simulink model "DABThermalAnalysisWithCustomMOSFET"  (R2026a)
settings: Solver=ode23t  StopTime=0.06  MaxStep=1e-5  AbsTol=1e-3
PreLoadFcn:
  | DABThermalAnalysisWithCustomMOSFETInputParameters;
model workspace (MAT data in the model file):
  ConverterKey = "DAB"
undefined symbols (not defined in the file): DAB, DABController, DABDesign, DiscIntNeverNeededParam, M1p, M1s, M2p, M2s, M3p, M3s, M4p, M4s
libraries: ee_lib x21, nesl_utility x16, fl_lib x11, slpidlib x4, simulink_extras x1
(part 1 of 2)
settings Model: SimulationMode=accelerator  Creator=vsolaise  LastModifiedBy=vsolaise
settings SimscapeCC: SimscapeNominalValues="[{\"value\":\"1\",\"unit\":\"A\"},{\"value\":\"1\",\"unit\":\"bar\"},{\"value\":\"1\",\"unit\":\"cm^2\"},{\"value\":\"1\",\"unit\":\"cm^3/s\"},{\"value\":\"1\",\"unit\":\"kJ/kg\"},{\"value\":\"1\",\"unit\":\"kW\"},{\"value\":\"1\",\"unit\":\"l\"},{\"value\":\"1\",\"unit\":\"N\"},{\"value\":\"1\",\"unit\":\"N*m\"},{\"value\":\"1\",\"unit\":\"V\"}]"  SimscapeLogName=simlogDABThermal  SimscapeLogDataHistory=5000.0

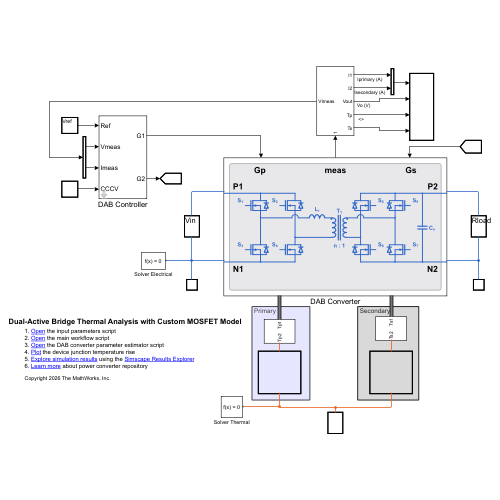
[thumbnail: Simulink's stored preview of the top-level diagram]
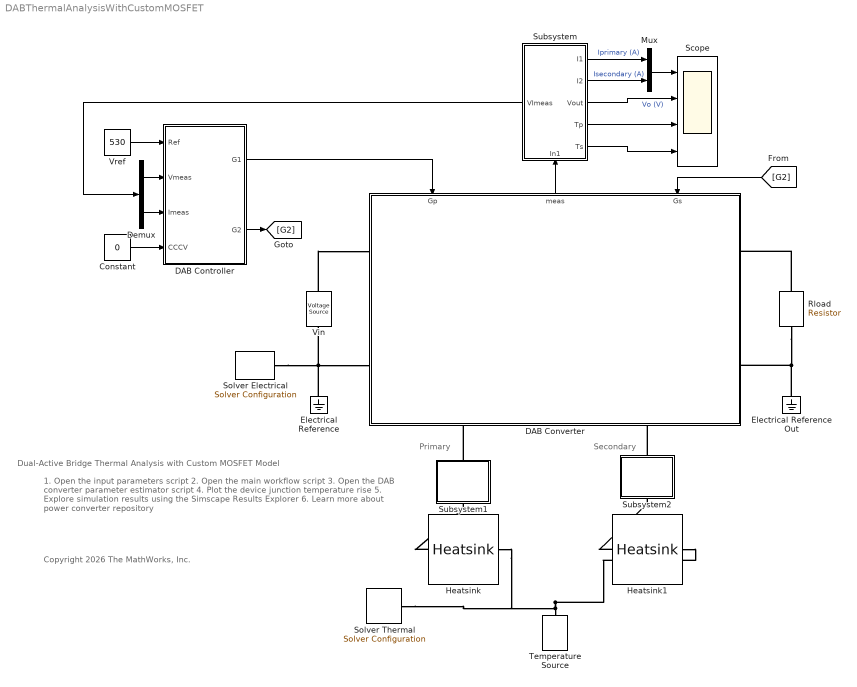
== system DABThermalAnalysisWithCustomMOSFET ==
  note: Secondary
  note: Primary
  note: Copyright 2026 The MathWorks, Inc.
  note: Dual-Active Bridge Thermal Analysis with Custom MOSFET Model
  note: 1. Open the input parameters script
      | 2. Open the main workflow script
      | 3. Open the DAB converter parameter estimator script
      | 4. Plot the device junction temperature rise
      | 5. Explore simulation results using the Simscape Results Explorer
      | 6. Learn more about power converter repository
  Constant : Constant  Value=0
  DAB Controller : Subsystem  mask(Dual Active Bridge Phase-Shift Controller){outputSelect=Gate Signals, cntrlSelect=PI controller (Continuous), Vbase=DABDesign.V2nom.value, Pbase=DABDesign.ratedPower.value, Fsw=DABDesign.switchingFrequency.value, Tdead=DABDesign.deadTime.value, primaryGateVoltage=DABController.gateVoltage, secondaryGateVoltage=DABController.gateVoltage, Ts=DABController.sampleTime, phaseShiftMax=DABController.phaseShiftMax, phaseShiftMin=DABController.phaseShiftMin, Kp=DABController.currentLoopProportionalGain, Ki=DABController.currentLoopIntegralGain, Kpv=DABController.voltageLoopProportionalGain, Kiv=DABController.voltageLoopIntegralGain}
      mask prompts: outputSelect "Output mode"; cntrlSelect "Controller type"; Vbase "Nominal output voltage (V)"; Pbase "Nominal power (W)"; Fsw "Switching frequency (Hz)"; Tdead "Dead time (s)"; primaryGateVoltage "Primary gate voltage (V)"; secondaryGateVoltage "Secondary gate voltage (V)"; Ts "Sample time (s)"; phaseShiftMax "Max phase shift (rad)"; phaseShiftMin "Min phase shift (rad)"; Kp "Proportional gain (current loop)"; Ki "Integral gain (current loop)"; Kpv "Proportional gain (voltage loop)"; Kiv "Integral gain (voltage loop)"
      mask help:
      | Phase-shift controller for the dual-active-bridge converter, in constant-current or constant-voltage mode. The CCCV input selects which loop runs: CC regulates Imeas against a current reference on Ref, normalized on the base current Pbase/Vbase; CV regulates Vmeas against a voltage reference on Ref, normalized on Vbase. Either PI drives the bridge-to-bridge phase shift, limited by phaseShiftMin and phaseShiftMax. Offers PI controllers in continuous or discrete form, with selectable phase shift or gate signal output.
      |
      | Outputs G1 and G2 are the primary and secondary bridge gate vectors, at the levels set by primaryGateVoltage and secondaryGateVoltage. In Phase Shift (rad) mode both outputs instead carry the phase shift itself, for use with an averaged plant.
      mask init:
      | dabControllerMaskInit(gcb);
      mask TypeOptions outputSelect: Gate Signals | Phase Shift (rad)
      mask Callback outputSelect: selectDABControllerOutputMode(gcb);
      mask TypeOptions cntrlSelect: PI controller (Continuous) | PI controller (Discrete)
      mask Callback cntrlSelect: selectDABControllerType(gcb);
      mask DialogControl Container5 Prompt: DAB Converter Parameter
      mask DialogControl ControllerPanel Prompt: Current Controller
      mask DialogControl VoltageLoopPanel Prompt: Voltage Controller
  DAB Converter : Subsystem
      settings: CopyFcn="set_param(gcbh,\"LinkStatus\",\"none\");"  PortSchema="{\"entries\":[{\"content\":{\"sides\":[{\"content\":{\"connectorIds\":[\"LConn1\",\"LConn2\"]},\"type\":\"ConnectorPlacement.EquallySpacedRectSide\",\"uuid\":\"033d868c-c914-47ac-88c6-7cc8bbca37ec\"},{\"content\":{\"connectorIds\":[\"RConn1\",\"RConn2\"],\"side\":\"RIGHT\"},\"type\":\"ConnectorPlacement.EquallySpacedRectSide\",\"uuid\":\"51ef52ad-95d3-4257-8134-5dc220f84f04\"},{\"content\":{\"connectorIds\":[\"In1\",\"Out1\",\"In2\"],\"side\":\"TOP\"},\"type\":\"ConnectorPlacement.EquallySpacedRectSide\",\"uuid\":\"aa7ed817-9ae7-4471-a537-30f60ddc8f94\"},{\"content\":{\"connectorIds\":[\"RConn3\",\"RConn4\"],\"side\":\"BOTTOM\"},\"type\":\"ConnectorPlacement.EquallySpacedRectSide\",\"uuid\":\"1eb7cc02-5c97-4e68-b623-57bf124e9704\"}]},\"type\":\"ConnectorPlacement.EquallySpacedConnector\",\"uuid\":\"613f6d24-3cc9-4a3f-99a5-466a272a8233\"}],\"packageUris\":[\"http://schema.mathworks.com/mf0/Connector/R2020b\"],\"version\":\"1.0\"}"
      mask Display: image('DABConverterIcon.svg');
  Demux : Demux  Outputs=2
  Electrical Reference : fl_lib/Electrical/Electrical Elements/Electrical Reference
  Electrical Reference Out : fl_lib/Electrical/Electrical Elements/Electrical Reference
  Heatsink : ee_lib/Passive/Thermal/Heatsink  parameterization=ee.enum.passive.thermal.heatsinkParam.datasheet  convection=ee.enum.passive.thermal.heatsinkConvection.natural  T_vec_Q=[10, 30, 50, 70, 90] K  v_vec_Q=[0, 1, 2, 3] m/s  Q_TLU1=[10, 30, 50, 70, 90]/DAB.HeatsinkPri.sinkToAmbientResistance W  Q_TLU2=[6.1, 18.8, 22.8, 25.7; 23.6, 61.1, 73, 81.5; 44.5, 106.4, 125.9, 140.1; 67.5, 153.5, 180.7, 200.3; 92.3, 202.1, 236.9, 262] W  T_vec_h=[10, 30, 50, 70, 90] K  v_vec_h=[0, 1, 2, 3] m/s  h_TLU1=[5.4, 7.02, 7.98, 8.68, 9.26] W/(K*m^2)  h_TLU2=[5.4, 17.86, 22.17, 25.41; 7.02, 19.49, 23.8, 27.03; 7.97, 20.44, 24.75, 27.99; 8.68, 21.15, 25.46, 28.69; 9.26, 21.73, 26.04, 29.27] W/(K*m^2)  h_vec=[5, 10, 15, 20, 25, 30] W/(K*m^2)  eff_TLU=[96.97, 94.16, 91.53, 89.08, 86.78, 84.62]  height=38.1e-3 m  thick=6.5e-4 m  depth=139.7e-3 m  gap=9.4e-3 m  num_fins=11  k_fin=237 W/(K*m)  A_total=0.1171 m^2  nu=1.51e-5 m^2/s  alpha=2.07e-5 m^2/s  k_fluid=25e-3 W/(K*m)  beta=3.3e-3 1/K  mass=DAB.HeatsinkPri.mass kg  sp_heat=DAB.HeatsinkPri.specificHeat J/(K*kg)  T_hs_specify=on  T_hs_priority=High  T_hs=DAB.HeatsinkPri.initialTemperature degC  T_hs_nominal_specify=off  T_hs_nominal_value=1  T_hs_nominal_unit=K  Q_A_specify=off  Q_A_priority=None  Q_A=0 W  Q_A_nominal_specify=off  Q_A_nominal_value=1  Q_A_nominal_unit=W  Q_C_specify=off  Q_C_priority=None  Q_C=0 W  Q_C_nominal_specify=off  Q_C_nominal_value=1  Q_C_nominal_unit=W
  Heatsink1 : ee_lib/Passive/Thermal/Heatsink  parameterization=ee.enum.passive.thermal.heatsinkParam.datasheet  convection=ee.enum.passive.thermal.heatsinkConvection.natural  T_vec_Q=[10, 30, 50, 70, 90] K  v_vec_Q=[0, 1, 2, 3] m/s  Q_TLU1=[10, 30, 50, 70, 90]/DAB.HeatsinkSec.sinkToAmbientResistance W  Q_TLU2=[6.1, 18.8, 22.8, 25.7; 23.6, 61.1, 73, 81.5; 44.5, 106.4, 125.9, 140.1; 67.5, 153.5, 180.7, 200.3; 92.3, 202.1, 236.9, 262] W  T_vec_h=[10, 30, 50, 70, 90] K  v_vec_h=[0, 1, 2, 3] m/s  h_TLU1=[5.4, 7.02, 7.98, 8.68, 9.26] W/(K*m^2)  h_TLU2=[5.4, 17.86, 22.17, 25.41; 7.02, 19.49, 23.8, 27.03; 7.97, 20.44, 24.75, 27.99; 8.68, 21.15, 25.46, 28.69; 9.26, 21.73, 26.04, 29.27] W/(K*m^2)  h_vec=[5, 10, 15, 20, 25, 30] W/(K*m^2)  eff_TLU=[96.97, 94.16, 91.53, 89.08, 86.78, 84.62]  height=38.1e-3 m  thick=6.5e-4 m  depth=139.7e-3 m  gap=9.4e-3 m  num_fins=11  k_fin=237 W/(K*m)  A_total=0.1171 m^2  nu=1.51e-5 m^2/s  alpha=2.07e-5 m^2/s  k_fluid=25e-3 W/(K*m)  beta=3.3e-3 1/K  mass=DAB.HeatsinkSec.mass kg  sp_heat=DAB.HeatsinkSec.specificHeat J/(K*kg)  T_hs_specify=on  T_hs_priority=High  T_hs=DAB.HeatsinkSec.initialTemperature degC  T_hs_nominal_specify=off  T_hs_nominal_value=1  T_hs_nominal_unit=K  Q_A_specify=off  Q_A_priority=None  Q_A=0 W  Q_A_nominal_specify=off  Q_A_nominal_value=1  Q_A_nominal_unit=W  Q_C_specify=off  Q_C_priority=None  Q_C=0 W  Q_C_nominal_specify=off  Q_C_nominal_value=1  Q_C_nominal_unit=W
  Mux : Mux  Inputs=2
  Rload : fl_lib/Electrical/Electrical Elements/Resistor  R=40 Ohm  i_specify=off  i_priority=None  i=0 A  i_nominal_specify=off  i_nominal_value=1  i_nominal_unit=A  v_specify=off  v_priority=None  v=0 V  v_nominal_specify=off  v_nominal_value=1  v_nominal_unit=V
  Scope : Scope  NumInputPorts=4
      settings: Title=Transformer current  ActiveDisplayYMinimum=-32.189332854725691  ActiveDisplayYMaximum=31.187175123208139  YLabel=Current (A)
  Solver Electrical : nesl_utility/Solver Configuration  PhysicalDomain=network_engine_domain  SubClassName=solver  LeftPortType=input  RightPortType=generic  Tones=[]  Harmonics=[]  SimulateNoise=off  Profile=off  UseLocalSampling=off  EnableSwitchedLinearOptims=on  FrequencyDomain=off  UseCCode=off  RelTol=0.001  AbsTol=0.001  MinStep=1e-09  ToWorkspace=off  RevertToSquareIcSolve=off  NumHomotopyIterations=100  PhasorMode=off  PhasorModeNumHarmonics=1  ConsistencySolver=NEWTON_XTOL_AFTER_FTOL  CanonicalOrdering=UNORDERED  OptimizeIntermediates=UNOPTIMIZED  IndexReductionMethod=DerivativeReplacement  DoDC=off  ResidualTolerance=1e-09  ConsistencyTolSource=GLOBAL  ConsistencyAbsTol=0.001  ConsistencyRelTol=0.001  ConsistencyTolFactor=0.001  UseLocalSolver=on  LocalSolverChoice=NE_PARTITIONING_ADVANCER  ResolveIndetEquations=on  FunctionEvalNumThread=1  LocalSolverSampleTime=1.5e-7  DoFixedCost=off  MaxNonlinIter=20  MaxModeIter=2  ComputeImpulses=off  ImpulseIterations=2  LinearAlgebra=auto  LinearAlgebraNumThread=0  EquationFormulation=NE_TIME_EF  DelaysMemoryBudget=1024  AutomaticFiltering=on  FilteringTimeConstant=0.001  PartitionStorageMethod=AS_NEEDED  PartitionMemoryBudget=1024  PartitionMethod=ROBUST  MultibodyUseLocalSolver=off  MultibodyLocalSolverChoice=ODE1  MultibodyLocalSolverSampleTime=0.001
  Solver Thermal : nesl_utility/Solver Configuration  PhysicalDomain=network_engine_domain  SubClassName=solver  LeftPortType=input  RightPortType=generic  Tones=[]  Harmonics=[]  SimulateNoise=off  Profile=off  UseLocalSampling=off  EnableSwitchedLinearOptims=on  FrequencyDomain=off  UseCCode=off  RelTol=0.001  AbsTol=0.001  MinStep=1e-09  ToWorkspace=off  RevertToSquareIcSolve=off  NumHomotopyIterations=100  PhasorMode=off  PhasorModeNumHarmonics=1  ConsistencySolver=NEWTON_XTOL_AFTER_FTOL  CanonicalOrdering=CANONICAL  OptimizeIntermediates=OPTIMIZED  IndexReductionMethod=DerivativeReplacement  DoDC=off  ResidualTolerance=1e-09  ConsistencyTolSource=GLOBAL  ConsistencyAbsTol=0.001  ConsistencyRelTol=0.001  ConsistencyTolFactor=0.001  UseLocalSolver=on  LocalSolverChoice=NE_BACKWARD_EULER_ADVANCER  ResolveIndetEquations=on  FunctionEvalNumThread=1  LocalSolverSampleTime=0.00001  DoFixedCost=off  MaxNonlinIter=3  MaxModeIter=2  ComputeImpulses=off  ImpulseIterations=2  LinearAlgebra=auto  LinearAlgebraNumThread=0  EquationFormulation=NE_TIME_EF  DelaysMemoryBudget=1024  AutomaticFiltering=on  FilteringTimeConstant=0.001  PartitionStorageMethod=AS_NEEDED  PartitionMemoryBudget=1024  PartitionMethod=ROBUST  MultibodyUseLocalSolver=off  MultibodyLocalSolverChoice=ODE1  MultibodyLocalSolverSampleTime=0.001
  Subsystem : Subsystem
      settings: PortSchema="{\"entries\":[{\"content\":{\"sides\":[{\"content\":{\"connectorIds\":[\"Out6\"]},\"type\":\"ConnectorPlacement.EquallySpacedRectSide\",\"uuid\":\"f2b899f7-a6f0-4063-b280-75fc43e532d5\"},{\"content\":{\"connectorIds\":[\"Out1\",\"Out2\",\"Out3\",\"Out4\",\"Out5\"],\"side\":\"RIGHT\"},\"type\":\"ConnectorPlacement.EquallySpacedRectSide\",\"uuid\":\"5de70531-a79e-4c62-9cd6-16ab34a78e6e\"},{\"content\":{\"side\":\"TOP\"},\"type\":\"ConnectorPlacement.EquallySpacedRectSide\",\"uuid\":\"e5bc4a57-59c4-404a-a3d7-aeb4f7590bd8\"},{\"content\":{\"connectorIds\":[\"In1\"],\"side\":\"BOTTOM\"},\"type\":\"ConnectorPlacement.EquallySpacedRectSide\",\"uuid\":\"d1dcebc2-7af2-4d54-9158-2e062e509fbc\"}]},\"type\":\"ConnectorPlacement.EquallySpacedConnector\",\"uuid\":\"ad567749-1bde-47d1-aaf1-1f8d8a2cad80\"}],\"packageUris\":[\"http://schema.mathworks.com/mf0/Connector/R2020b\"],\"version\":\"1.0\"}"
  Subsystem1 : Subsystem
  Subsystem2 : Subsystem
  Temperature Source : fl_lib/Thermal/Thermal Sources/Temperature Source  temperature=298.15 K
  Vin : ee_lib/Sources/Voltage Source  dc_voltage=770 V  ac_voltage=0 V  ac_shift=0 rad  ac_frequency=60 Hz  noise_mode=ee.enum.sources.noise.Disabled  PSD=0 V^2/Hz  sample_time=1e-3 s  repeatability=ee.enum.sources.repeatability.NotRepeatable  user_seed=0  auto_seed=1556750757  i_specify=off  i_priority=None  i=0 A  i_nominal_specify=off  i_nominal_value=1  i_nominal_unit=A  v_specify=off  v_priority=None  v=0 V  v_nominal_specify=off  v_nominal_value=1  v_nominal_unit=V
  Vref : Constant  Value=530
  wires:
  DAB Controller/2(G2) -> [G2]
  Constant/1 -> DAB Controller/4(CCCV)
  Subsystem/1(I1) -> Mux/1  "Iprimary (A)"
  Subsystem/2(I2) -> Mux/2  "Isecondary (A)"
  DAB Converter/1(meas) -> Subsystem/1(In1)
  Vref/1 -> DAB Controller/1(Ref)
  Demux/2 -> DAB Controller/3(Imeas)
  Demux/1 -> DAB Controller/2(Vmeas)
  Subsystem/6(VImeas) -> Demux/1
  DAB Controller/1(G1) -> DAB Converter/1(Gp)
  [G2] -> DAB Converter/2(Gs)
  Mux/1 -> Scope/1
  Subsystem/3(Vout) -> Scope/2  "Vo (V)"
  Subsystem/4(Tp) -> Scope/3
  Subsystem/5(Ts) -> Scope/4
  connections:
  Vin/LConn1 -- DAB Converter/LConn1
  Rload/LConn1 -- DAB Converter/RConn1
  Solver Electrical/RConn1 -- Electrical Reference/LConn1 -- Vin/RConn1 -- DAB Converter/LConn2
  Rload/RConn1 -- Electrical Reference Out/LConn1 -- DAB Converter/RConn2
  Temperature Source/LConn1 -- Heatsink1/LConn1 -- Heatsink/LConn1 -- Solver Thermal/RConn1
  Subsystem2/RConn1 -- DAB Converter/RConn4
  Subsystem1/RConn1 -- DAB Converter/RConn3
  Heatsink1/RConn1 -- Subsystem2/LConn1
  Heatsink/RConn1 -- Subsystem1/LConn1

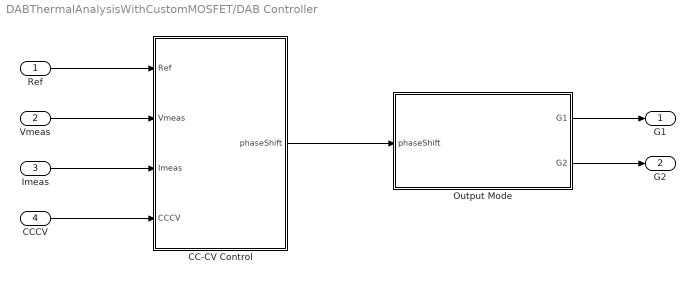
== system DABThermalAnalysisWithCustomMOSFET/DAB Controller ==
  Ref : Inport
  Vmeas : Inport  Port=2
  Imeas : Inport  Port=3
  CCCV : Inport  Port=4
  CC-CV Control : Subsystem
  Output Mode : Subsystem  Variant=on  VariantControlMode=label  LabelModeActiveChoice=PWMSignal
  G1 : Outport
  G2 : Outport  Port=2
  wires:
  CCCV/1 -> CC-CV Control/4(CCCV)
  Imeas/1 -> CC-CV Control/3(Imeas)
  Vmeas/1 -> CC-CV Control/2(Vmeas)
  Ref/1 -> CC-CV Control/1(Ref)
  Output Mode/2(G2) -> G2/1
  Output Mode/1(G1) -> G1/1
  CC-CV Control/1(phaseShift) -> Output Mode/1(phaseShift)

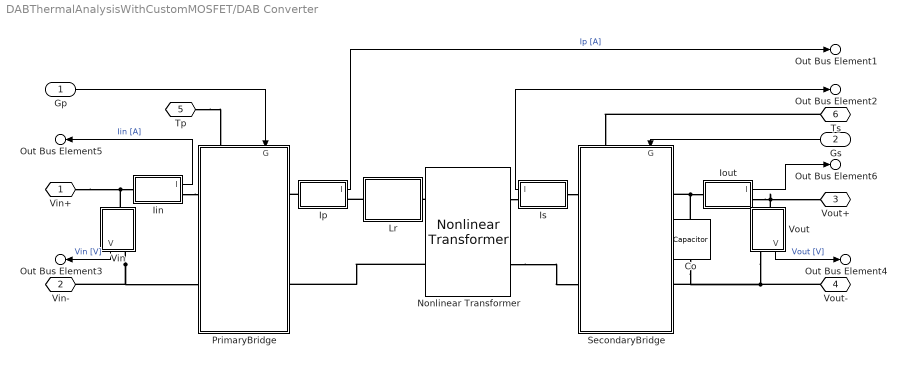
== system DABThermalAnalysisWithCustomMOSFET/DAB Converter ==
  Gp : Inport
  Gs : Inport  Port=2
  Co : ee_lib/Passive/Capacitor  cap_option=ee.enum.passive.capacitor.capOption.const  c=DAB.Co F  Cvec=[1e-05, 1e-06] F  Vvec=[0, 10] V  CV_table_symmetry=ee.enum.passive.capacitor.tableSymmetry.yes  f_vec=[1, 10] kHz  DFext_vec=[.8, 1.2]  enable_C_tol=ee.enum.toleranceApplication.none  averaging_period=0 s  C_tol=5  tol_distribution=ee.enum.toleranceDistribution.uniform  nSigma=4  r=DAB.Rco Ohm  g=0 1/Ohm  enable_operating_limits=ee.enum.enable.no  operating_limit_action=ee.enum.passive.reportOpLim.warn  max_working_voltage_range=[-25, 25] V  power_rating=1 W  maxTemperature=85 degC  thermalEnable=false  thermalMass=1 J/K  i_specify=off  i_priority=None  i=0 A  i_nominal_specify=off  i_nominal_value=1  i_nominal_unit=A  v_specify=off  v_priority=None  v=0 V  v_nominal_specify=off  v_nominal_value=1  v_nominal_unit=V  vc_specify=on  vc_priority=High  vc=DAB.Vco V  vc_nominal_specify=off  vc_nominal_value=1  vc_nominal_unit=V  T_specify=off  T_priority=None  T=298.15 K  T_nominal_specify=off  T_nominal_value=1  T_nominal_unit=K
  Iin : Subsystem
      mask Display: disp('I')
  Iout : Subsystem
      mask Display: disp('I')
  Ip : Subsystem
      mask Display: disp('I')
  Is : Subsystem
      settings: PortSchema="{\"entries\":[{\"content\":{\"sides\":[{\"content\":{\"connectorIds\":[\"Out1\",\"LConn1\"]},\"type\":\"ConnectorPlacement.EquallySpacedRectSide\",\"uuid\":\"da66b42d-39ba-4e5d-9b19-dc680792542d\"},{\"content\":{\"connectorIds\":[\"RConn1\"],\"side\":\"RIGHT\"},\"type\":\"ConnectorPlacement.EquallySpacedRectSide\",\"uuid\":\"9a34d54a-b1f0-405a-82c9-4333c7864e33\"},{\"content\":{\"side\":\"TOP\"},\"type\":\"ConnectorPlacement.EquallySpacedRectSide\",\"uuid\":\"3d98f795-d173-4072-aa84-47617691d0d7\"}]},\"type\":\"ConnectorPlacement.EquallySpacedConnector\",\"uuid\":\"cc1a3107-18f6-4c4b-a82f-56637250e4a4\"}],\"packageUris\":[\"http://schema.mathworks.com/mf0/Connector/R2020b\"],\"version\":\"1.0\"}"
      mask Display: disp('I')
  Lr : Subsystem
  Nonlinear Transformer : ee_lib/Passive/Transformers/Nonlinear Transformer  Nw=DAB.turnsRatio  Nw2=1  winding_param_option=2  Req=0 Ohm  Leq=0 H  R_1=DAB.RLlk1 Ohm  L_1=DAB.Llk1 H  R_2=DAB.RLlk2 Ohm  L_2=DAB.Llk2 H  averaging_period=0 s  R_m=15000 Ohm  parameterization_option=1  H_data=[0, 200, 400, 600, 800, 1000] A/m  B_data=[0, .81, 1.25, 1.42, 1.48, 1.49] T  length_effective=0.2 m  area_effective=2e-4 m^2  L=DAB.Lm H  L_sat=1e-2 H  current_data=[0, .4, .8, 1.2, 1.6, 2] A  magnetic_flux_data=[0, .161, .25, .284, .295, .299] .* 1e-3 Wb  magnetic_flux_sat=1.6e-04 Wb  dBdH0=0.005 T*m/A  B1=1.49 T  H1=1000 A/m  c=0.1  K=200 A/m  alpha=1e-4  interpolation_option=1  Leq_i0=0 A  L1_i0=0 A  L2_i0=0 A  x0_option=1  i_L0=0 A  phi0=0 Wb  B0=0 T  H0=0 A/m  Leq_g=1e-9 1/Ohm  L1_g=1e-9 1/Ohm  L2_g=1e-9 1/Ohm
  PrimaryBridge : Subsystem
      settings: PortSchema="{\"entries\":[{\"content\":{\"sides\":[{\"content\":{\"connectorIds\":[\"LConn1\",\"LConn2\"]},\"type\":\"ConnectorPlacement.EquallySpacedRectSide\",\"uuid\":\"749830e9-51d7-44b2-bde2-4b1703907a46\"},{\"content\":{\"connectorIds\":[\"RConn1\",\"RConn2\"],\"side\":\"RIGHT\"},\"type\":\"ConnectorPlacement.EquallySpacedRectSide\",\"uuid\":\"8c887d8f-8aba-48f0-8b02-913eb5d6f212\"},{\"content\":{\"connectorIds\":[\"LConn3\",\"In1\"],\"side\":\"TOP\"},\"type\":\"ConnectorPlacement.EquallySpacedRectSide\",\"uuid\":\"cac777da-3cda-42c9-9648-d6d8ad2054e0\"}]},\"type\":\"ConnectorPlacement.EquallySpacedConnector\",\"uuid\":\"f342ee6c-a4b8-476e-aaf5-48ac9419b143\"}],\"packageUris\":[\"http://schema.mathworks.com/mf0/Connector/R2020b\"],\"version\":\"1.0\"}"
  SecondaryBridge : Subsystem
      settings: PortSchema="{\"entries\":[{\"content\":{\"sides\":[{\"content\":{\"connectorIds\":[\"LConn1\",\"LConn2\"]},\"type\":\"ConnectorPlacement.EquallySpacedRectSide\",\"uuid\":\"749830e9-51d7-44b2-bde2-4b1703907a46\"},{\"content\":{\"connectorIds\":[\"RConn1\",\"RConn2\"],\"side\":\"RIGHT\"},\"type\":\"ConnectorPlacement.EquallySpacedRectSide\",\"uuid\":\"8c887d8f-8aba-48f0-8b02-913eb5d6f212\"},{\"content\":{\"connectorIds\":[\"In1\",\"LConn3\"],\"side\":\"TOP\"},\"type\":\"ConnectorPlacement.EquallySpacedRectSide\",\"uuid\":\"cac777da-3cda-42c9-9648-d6d8ad2054e0\"}]},\"type\":\"ConnectorPlacement.EquallySpacedConnector\",\"uuid\":\"f342ee6c-a4b8-476e-aaf5-48ac9419b143\"}],\"packageUris\":[\"http://schema.mathworks.com/mf0/Connector/R2020b\"],\"version\":\"1.0\"}"
  Vin : Subsystem
      mask Display: disp('V')
  Vout : Subsystem
      settings: PortSchema="{\"entries\":[{\"content\":{\"sides\":[{\"content\":{\"connectorIds\":[\"LConn1\"]},\"type\":\"ConnectorPlacement.EquallySpacedRectSide\",\"uuid\":\"da66b42d-39ba-4e5d-9b19-dc680792542d\"},{\"content\":{\"connectorIds\":[\"RConn1\",\"Out1\"],\"side\":\"RIGHT\"},\"type\":\"ConnectorPlacement.EquallySpacedRectSide\",\"uuid\":\"9a34d54a-b1f0-405a-82c9-4333c7864e33\"},{\"content\":{\"side\":\"TOP\"},\"type\":\"ConnectorPlacement.EquallySpacedRectSide\",\"uuid\":\"3d98f795-d173-4072-aa84-47617691d0d7\"}]},\"type\":\"ConnectorPlacement.EquallySpacedConnector\",\"uuid\":\"cc1a3107-18f6-4c4b-a82f-56637250e4a4\"}],\"packageUris\":[\"http://schema.mathworks.com/mf0/Connector/R2020b\"],\"version\":\"1.0\"}"
      mask Display: disp('V')
  Vin+ : PMIOPort  Side=Left
  Vin- : PMIOPort  Port=2  Side=Left
  Vout+ : PMIOPort  Port=3  Side=Right
  Vout- : PMIOPort  Port=4  Side=Right
  Tp : PMIOPort  Port=5  Side=Right
  Ts : PMIOPort  Port=6  Side=Right
  Out Bus Element1 : Outport  PortName=meas  Element=Ip [A]
  Out Bus Element2 : Outport  PortName=meas  Element=Is [A]
  Out Bus Element3 : Outport  PortName=meas  Element=Vin [V]
  Out Bus Element4 : Outport  PortName=meas  Element=Vout [V]
  Out Bus Element5 : Outport  PortName=meas  Element=Iin [A]
  Out Bus Element6 : Outport  PortName=meas  Element=Iout [A]
  wires:
  Iin/1(I) -> Out Bus Element5/1  "Iin [A]"
  Gp/1 -> PrimaryBridge/1(G)
  Vin/1(V) -> Out Bus Element3/1  "Vin [V]"
  Iout/1(I) -> Out Bus Element6/1
  Vout/1(V) -> Out Bus Element4/1  "Vout [V]"
  Ip/1(I) -> Out Bus Element1/1  "Ip [A]"
  Is/1(I) -> Out Bus Element2/1
  Gs/1 -> SecondaryBridge/1(G)
  connections:
  Vin/RConn1 -- Vin-/RConn1 -- PrimaryBridge/LConn2
  Vin+/RConn1 -- Vin/LConn1 -- Iin/LConn1
  Vout/LConn1 -- Vout+/RConn1 -- Iout/RConn1
  Vout-/RConn1 -- Vout/RConn1 -- Co/RConn1 -- SecondaryBridge/LConn2
  Co/LConn1 -- Iout/LConn1 -- SecondaryBridge/LConn1
  Ip/LConn1 -- PrimaryBridge/RConn1
  Nonlinear Transformer/RConn2 -- SecondaryBridge/RConn2
  Iin/RConn1 -- PrimaryBridge/LConn1
  Nonlinear Transformer/LConn2 -- PrimaryBridge/RConn2
  Nonlinear Transformer/RConn1 -- Is/LConn1
  Lr/LConn1 -- Ip/RConn1
  Nonlinear Transformer/LConn1 -- Lr/RConn1
  Is/RConn1 -- SecondaryBridge/RConn1
  Tp/RConn1 -- PrimaryBridge/LConn3
  Ts/RConn1 -- SecondaryBridge/LConn3

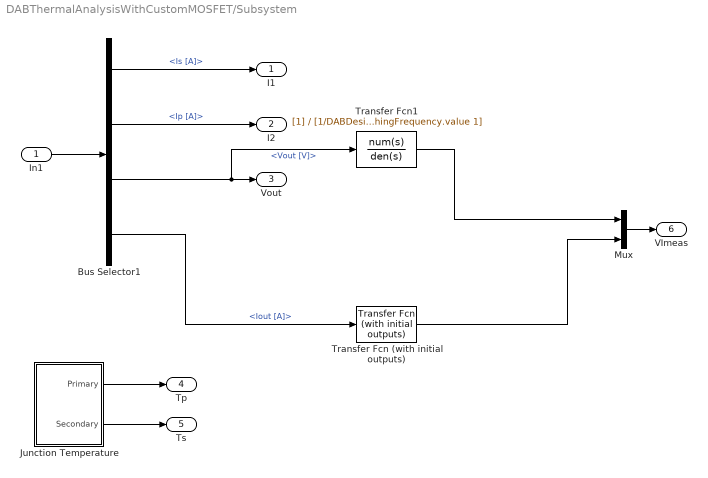
== system DABThermalAnalysisWithCustomMOSFET/Subsystem ==
  In1 : Inport
  Bus Selector1 : BusSelector  OutputSignals=Is [A],Ip [A],Vout [V],Iout [A]
  Junction Temperature : Subsystem
  Mux : Mux  Inputs=2
  Transfer Fcn (with initial outputs) : simulink_extras/Additional Linear/Transfer Fcn (with initial outputs)  N=[1]  D=[1/DABDesign.switchingFrequency.value 1]  Y0=DABDesign.V2nom.value  U0=DABDesign.V2nom.value
  Transfer Fcn1 : TransferFcn  Denominator=[1/DABDesign.switchingFrequency.value 1]
  I1 : Outport
  I2 : Outport  Port=2
  Vout : Outport  Port=3
  Tp : Outport  Port=4
  Ts : Outport  Port=5
  VImeas : Outport  Port=6
  wires:
  In1/1 -> Bus Selector1/1
  Bus Selector1/1 -> I1/1  "<Is [A]>"
  Bus Selector1/2 -> I2/1  "<Ip [A]>"
  Bus Selector1/3 -> Transfer Fcn1/1, Vout/1  "<Vout [V]>"
  Bus Selector1/4 -> Transfer Fcn (with initial outputs)/1  "<Iout [A]>"
  Transfer Fcn (with initial outputs)/1 -> Mux/2
  Transfer Fcn1/1 -> Mux/1
  Mux/1 -> VImeas/1
  Junction Temperature/1(Primary) -> Tp/1
  Junction Temperature/2(Secondary) -> Ts/1

== system DABThermalAnalysisWithCustomMOSFET/Subsystem1 ==
  Simscape Bus : SimscapeBus  HierarchyStrings=M1p;M2p;M3p;M4p
  Thermal Resistor{,1..3} (4 alike) : ee_lib/Passive/Thermal/Thermal Resistor  R=DAB.caseToSinkResistance K/W  T_specify=off  T_priority=None  T=0 K  T_nominal_specify=off  T_nominal_value=1  T_nominal_unit=K  Q_specify=off  Q_priority=None  Q=0 W  Q_nominal_specify=off  Q_nominal_value=1  Q_nominal_unit=W
  Tp1 : PMIOPort  Side=Right
  Tp2 : PMIOPort  Port=2  Side=Left
  connections:
  Thermal Resistor3/LConn1 -- Simscape Bus/LConn4
  Thermal Resistor2/LConn1 -- Simscape Bus/LConn3
  Thermal Resistor1/LConn1 -- Simscape Bus/LConn2
  Thermal Resistor/LConn1 -- Simscape Bus/LConn1
  Simscape Bus/RConn1 -- Tp1/RConn1
  Thermal Resistor3/RConn1 -- Thermal Resistor2/RConn1 -- Thermal Resistor1/RConn1 -- Thermal Resistor/RConn1 -- Tp2/RConn1

== system DABThermalAnalysisWithCustomMOSFET/Subsystem2 ==
  Simscape Bus1 : SimscapeBus  HierarchyStrings=M1s;M2s;M3s;M4s
  Thermal Resistor{4..7} (4 alike) : ee_lib/Passive/Thermal/Thermal Resistor  R=DAB.caseToSinkResistance K/W  T_specify=off  T_priority=None  T=0 K  T_nominal_specify=off  T_nominal_value=1  T_nominal_unit=K  Q_specify=off  Q_priority=None  Q=0 W  Q_nominal_specify=off  Q_nominal_value=1  Q_nominal_unit=W
  Ts1 : PMIOPort  Side=Right
  Ts2 : PMIOPort  Port=2  Side=Left
  connections:
  Thermal Resistor7/LConn1 -- Simscape Bus1/LConn4
  Thermal Resistor6/LConn1 -- Simscape Bus1/LConn3
  Thermal Resistor7/RConn1 -- Thermal Resistor6/RConn1 -- Thermal Resistor4/RConn1 -- Thermal Resistor5/RConn1 -- Ts2/RConn1
  Thermal Resistor5/LConn1 -- Simscape Bus1/LConn2
  Thermal Resistor4/LConn1 -- Simscape Bus1/LConn1
  Simscape Bus1/RConn1 -- Ts1/RConn1

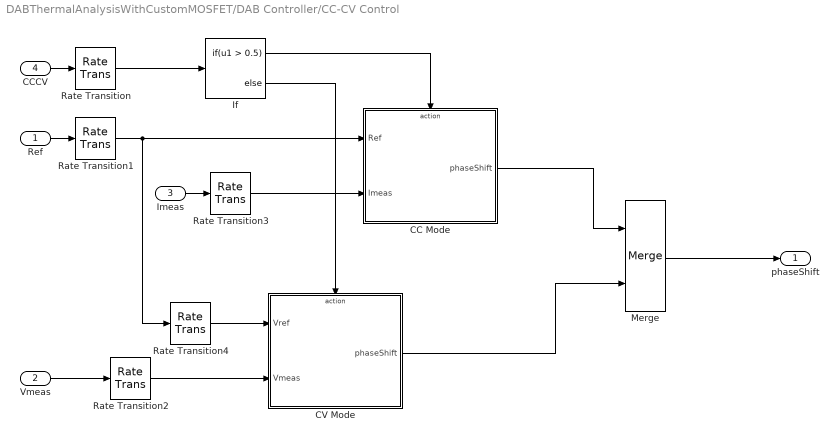
== system DABThermalAnalysisWithCustomMOSFET/DAB Controller/CC-CV Control ==
  Ref : Inport
  Vmeas : Inport  Port=2
  Imeas : Inport  Port=3
  CCCV : Inport  Port=4
  CC Mode : Subsystem  TreatAsAtomicUnit=on
  CV Mode : Subsystem  TreatAsAtomicUnit=on
  If : If  IfExpression=u1 > 0.5
  Merge : Merge
  Rate Transition{,1..4} (5 alike) : RateTransition
  phaseShift : Outport
  wires:
  Rate Transition2/1 -> CV Mode/2(Vmeas)
  Rate Transition1/1 -> CC Mode/1(Ref), Rate Transition4/1
  Rate Transition/1 -> If/1
  Imeas/1 -> Rate Transition3/1
  Vmeas/1 -> Rate Transition2/1
  Ref/1 -> Rate Transition1/1
  If/2 -> CV Mode/Action
  If/1 -> CC Mode/Action
  CCCV/1 -> Rate Transition/1
  Rate Transition3/1 -> CC Mode/2(Imeas)
  Merge/1 -> phaseShift/1
  CV Mode/1(phaseShift) -> Merge/2
  CC Mode/1(phaseShift) -> Merge/1
  Rate Transition4/1 -> CV Mode/1(Vref)

== system DABThermalAnalysisWithCustomMOSFET/DAB Controller/Output Mode ==
  phaseShift : Inport
  DutyCycle : Subsystem  VariantControl=DutyCycle
  PWMSignal : Subsystem  VariantControl=PWMSignal
  G1 : Outport
  G2 : Outport  Port=2

== system DABThermalAnalysisWithCustomMOSFET/DAB Converter/Iin ==
  Current Sensor : fl_lib/Electrical/Electrical Sensors/Current Sensor
  PS-Simulink Converter : nesl_utility/PS-Simulink Converter  PhysicalDomain=network_engine_domain  SubClassName=ps_output  LeftPortType=input  RightPortType=output  PseudoPeriodic=off  Frequencies=[]  VectorFormat=inherit  Unit=inherit  AffineConversion=off
  + : PMIOPort  Side=Left
  - : PMIOPort  Port=2  Side=Right
  I : Outport
  wires:
  PS-Simulink Converter/1 -> I/1
  connections:
  +/RConn1 -- Current Sensor/LConn1
  Current Sensor/RConn2 -- -/RConn1
  Current Sensor/RConn1 -- PS-Simulink Converter/LConn1

== system DABThermalAnalysisWithCustomMOSFET/DAB Converter/Iout ==
  Current Sensor : fl_lib/Electrical/Electrical Sensors/Current Sensor
  PS-Simulink Converter : nesl_utility/PS-Simulink Converter  PhysicalDomain=network_engine_domain  SubClassName=ps_output  LeftPortType=input  RightPortType=output  PseudoPeriodic=off  Frequencies=[]  VectorFormat=inherit  Unit=inherit  AffineConversion=off
  + : PMIOPort  Side=Left
  - : PMIOPort  Port=2  Side=Right
  I : Outport
  wires:
  PS-Simulink Converter/1 -> I/1
  connections:
  +/RConn1 -- Current Sensor/LConn1
  Current Sensor/RConn2 -- -/RConn1
  Current Sensor/RConn1 -- PS-Simulink Converter/LConn1

== system DABThermalAnalysisWithCustomMOSFET/DAB Converter/Ip ==
  Current Sensor : fl_lib/Electrical/Electrical Sensors/Current Sensor
  PS-Simulink Converter : nesl_utility/PS-Simulink Converter  PhysicalDomain=network_engine_domain  SubClassName=ps_output  LeftPortType=input  RightPortType=output  PseudoPeriodic=off  Frequencies=[]  VectorFormat=inherit  Unit=inherit  AffineConversion=off
  + : PMIOPort  Side=Left
  - : PMIOPort  Port=2  Side=Right
  I : Outport
  wires:
  PS-Simulink Converter/1 -> I/1
  connections:
  +/RConn1 -- Current Sensor/LConn1
  Current Sensor/RConn2 -- -/RConn1
  Current Sensor/RConn1 -- PS-Simulink Converter/LConn1

== system DABThermalAnalysisWithCustomMOSFET/DAB Converter/Is ==
  Current Sensor : fl_lib/Electrical/Electrical Sensors/Current Sensor
  PS-Simulink Converter : nesl_utility/PS-Simulink Converter  PhysicalDomain=network_engine_domain  SubClassName=ps_output  LeftPortType=input  RightPortType=output  PseudoPeriodic=off  Frequencies=[]  VectorFormat=inherit  Unit=inherit  AffineConversion=off
  + : PMIOPort  Side=Left
  - : PMIOPort  Port=2  Side=Right
  I : Outport
  wires:
  PS-Simulink Converter/1 -> I/1
  connections:
  +/RConn1 -- Current Sensor/LConn1
  Current Sensor/RConn2 -- -/RConn1
  Current Sensor/RConn1 -- PS-Simulink Converter/LConn1

== system DABThermalAnalysisWithCustomMOSFET/DAB Converter/Lr ==
  ExternalInductance : Subsystem
  P : PMIOPort  Side=Left
  N : PMIOPort  Port=2  Side=Right
  connections:
  P/RConn1 -- ExternalInductance/LConn1
  N/RConn1 -- ExternalInductance/RConn1

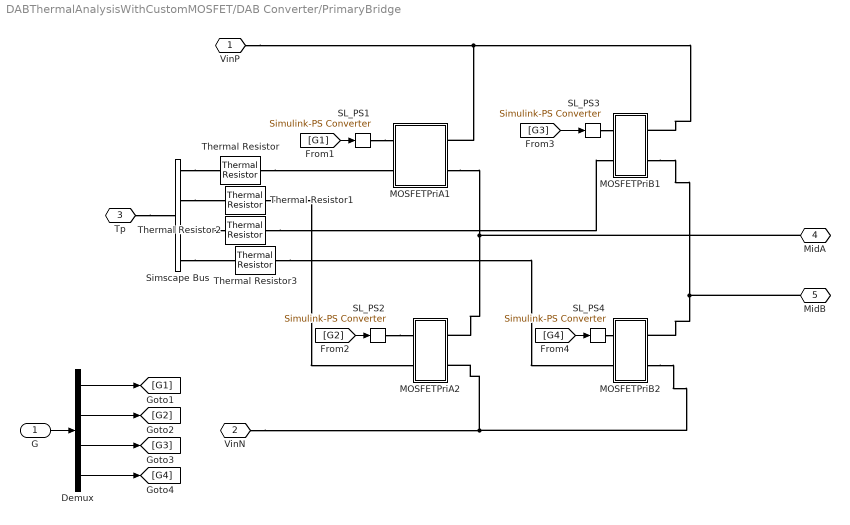
== system DABThermalAnalysisWithCustomMOSFET/DAB Converter/PrimaryBridge ==
  G : Inport
  Demux : Demux
  MOSFETPriA1 : Subsystem  ReferencedSubsystem=DABPrimaryMOSFETDevice
  MOSFETPriA2 : Subsystem  ReferencedSubsystem=DABPrimaryMOSFETDevice
  MOSFETPriB1 : Subsystem  ReferencedSubsystem=DABPrimaryMOSFETDevice
  MOSFETPriB2 : Subsystem  ReferencedSubsystem=DABPrimaryMOSFETDevice
  SL_PS{1..4} (4 alike) : nesl_utility/Simulink-PS Converter  PhysicalDomain=network_engine_domain  SubClassName=ps_input  LeftPortType=input  RightPortType=output  PseudoPeriodic=off  Frequencies=[]  NoiseDistribution=none  NoiseParameters=[]  Unit=1  AffineConversion=off  FilteringAndDerivatives=provide  SimscapeFilterOrder=1  InputFilterTimeConstant=0.001  UdotUserProvided=0
  Simscape Bus : SimscapeBus  HierarchyStrings=M1p;M2p;M3p;M4p
  Thermal Resistor{,1..3} (4 alike) : ee_lib/Passive/Thermal/Thermal Resistor  R=1e-3 K/W  T_specify=off  T_priority=None  T=0 K  T_nominal_specify=off  T_nominal_value=1  T_nominal_unit=K  Q_specify=off  Q_priority=None  Q=0 W  Q_nominal_specify=off  Q_nominal_value=1  Q_nominal_unit=W
  VinP : PMIOPort  Side=Left
  VinN : PMIOPort  Port=2  Side=Left
  Tp : PMIOPort  Port=3  Side=Left
  MidA : PMIOPort  Port=4  Side=Right
  MidB : PMIOPort  Port=5  Side=Right
  wires:
  Demux/3 -> [G3]
  [G2] -> SL_PS2/1
  [G4] -> SL_PS4/1
  G/1 -> Demux/1
  Demux/4 -> [G4]
  [G3] -> SL_PS3/1
  Demux/2 -> [G2]
  [G1] -> SL_PS1/1
  Demux/1 -> [G1]
  connections:
  MOSFETPriA1/RConn1 -- VinP/RConn1 -- MOSFETPriB1/RConn1
  MOSFETPriA2/RConn2 -- MOSFETPriB2/RConn2 -- VinN/RConn1
  MOSFETPriB2/RConn1 -- MOSFETPriB1/RConn2 -- MidB/RConn1
  MOSFETPriA1/RConn2 -- MidA/RConn1 -- MOSFETPriA2/RConn1
  SL_PS4/RConn1 -- MOSFETPriB2/LConn1
  SL_PS3/RConn1 -- MOSFETPriB1/LConn1
  SL_PS2/RConn1 -- MOSFETPriA2/LConn1
  SL_PS1/RConn1 -- MOSFETPriA1/LConn1
  Tp/RConn1 -- Simscape Bus/RConn1
  Thermal Resistor/RConn1 -- MOSFETPriA1/LConn2
  Thermal Resistor1/RConn1 -- MOSFETPriA2/LConn2
  Thermal Resistor2/RConn1 -- MOSFETPriB1/LConn2
  Thermal Resistor3/RConn1 -- MOSFETPriB2/LConn2
  Simscape Bus/LConn1 -- Thermal Resistor/LConn1
  Simscape Bus/LConn2 -- Thermal Resistor1/LConn1
  Simscape Bus/LConn3 -- Thermal Resistor2/LConn1
  Simscape Bus/LConn4 -- Thermal Resistor3/LConn1

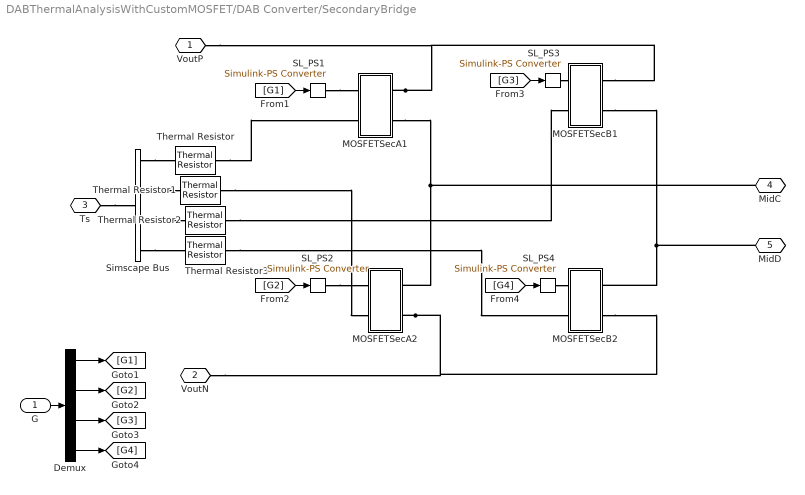
== system DABThermalAnalysisWithCustomMOSFET/DAB Converter/SecondaryBridge ==
  G : Inport
  Demux : Demux
  MOSFETSecA1 : Subsystem  ReferencedSubsystem=DABSecondaryMOSFETDevice
  MOSFETSecA2 : Subsystem  ReferencedSubsystem=DABSecondaryMOSFETDevice
  MOSFETSecB1 : Subsystem  ReferencedSubsystem=DABSecondaryMOSFETDevice
  MOSFETSecB2 : Subsystem  ReferencedSubsystem=DABSecondaryMOSFETDevice
  SL_PS{1..4} (4 alike) : nesl_utility/Simulink-PS Converter  PhysicalDomain=network_engine_domain  SubClassName=ps_input  LeftPortType=input  RightPortType=output  PseudoPeriodic=off  Frequencies=[]  NoiseDistribution=none  NoiseParameters=[]  Unit=1  AffineConversion=off  FilteringAndDerivatives=provide  SimscapeFilterOrder=1  InputFilterTimeConstant=0.001  UdotUserProvided=0
  Simscape Bus : SimscapeBus  HierarchyStrings=M1s;M2s;M3s;M4s
  Thermal Resistor{,1..3} (4 alike) : ee_lib/Passive/Thermal/Thermal Resistor  R=1e-3 K/W  T_specify=off  T_priority=None  T=0 K  T_nominal_specify=off  T_nominal_value=1  T_nominal_unit=K  Q_specify=off  Q_priority=None  Q=0 W  Q_nominal_specify=off  Q_nominal_value=1  Q_nominal_unit=W
  VoutP : PMIOPort  Side=Left
  VoutN : PMIOPort  Port=2  Side=Left
  Ts : PMIOPort  Port=3  Side=Left
  MidC : PMIOPort  Port=4  Side=Right
  MidD : PMIOPort  Port=5  Side=Right
  wires:
  Demux/2 -> [G2]
  Demux/4 -> [G4]
  Demux/3 -> [G3]
  G/1 -> Demux/1
  [G2] -> SL_PS2/1
  [G3] -> SL_PS3/1
  [G1] -> SL_PS1/1
  [G4] -> SL_PS4/1
  Demux/1 -> [G1]
  connections:
  MOSFETSecA1/RConn1 -- MOSFETSecB1/RConn1 -- VoutP/RConn1
  MOSFETSecA2/RConn2 -- MOSFETSecB2/RConn2 -- VoutN/RConn1
  MOSFETSecA1/RConn2 -- MidC/RConn1 -- MOSFETSecA2/RConn1
  MOSFETSecB1/RConn2 -- MidD/RConn1 -- MOSFETSecB2/RConn1
  SL_PS4/RConn1 -- MOSFETSecB2/LConn1
  SL_PS3/RConn1 -- MOSFETSecB1/LConn1
  SL_PS1/RConn1 -- MOSFETSecA1/LConn1
  SL_PS2/RConn1 -- MOSFETSecA2/LConn1
  Ts/RConn1 -- Simscape Bus/RConn1
  Simscape Bus/LConn2 -- Thermal Resistor1/LConn1
  Simscape Bus/LConn1 -- Thermal Resistor/LConn1
  Thermal Resistor2/RConn1 -- MOSFETSecB1/LConn2
  Simscape Bus/LConn4 -- Thermal Resistor3/LConn1
  Thermal Resistor/RConn1 -- MOSFETSecA1/LConn2
  Thermal Resistor1/RConn1 -- MOSFETSecA2/LConn2
  Simscape Bus/LConn3 -- Thermal Resistor2/LConn1
  Thermal Resistor3/RConn1 -- MOSFETSecB2/LConn2

== system DABThermalAnalysisWithCustomMOSFET/DAB Converter/Vin ==
  PS-Simulink Converter : nesl_utility/PS-Simulink Converter  PhysicalDomain=network_engine_domain  SubClassName=ps_output  LeftPortType=input  RightPortType=output  PseudoPeriodic=off  Frequencies=[]  VectorFormat=inherit  Unit=inherit  AffineConversion=off
  Voltage Sensor : fl_lib/Electrical/Electrical Sensors/Voltage Sensor
  + : PMIOPort  Side=Left
  - : PMIOPort  Port=2  Side=Right
  V : Outport
  wires:
  PS-Simulink Converter/1 -> V/1
  connections:
  +/RConn1 -- Voltage Sensor/LConn1
  Voltage Sensor/RConn2 -- -/RConn1
  Voltage Sensor/RConn1 -- PS-Simulink Converter/LConn1

== system DABThermalAnalysisWithCustomMOSFET/DAB Converter/Vout ==
  PS-Simulink Converter : nesl_utility/PS-Simulink Converter  PhysicalDomain=network_engine_domain  SubClassName=ps_output  LeftPortType=input  RightPortType=output  PseudoPeriodic=off  Frequencies=[]  VectorFormat=inherit  Unit=inherit  AffineConversion=off
  Voltage Sensor : fl_lib/Electrical/Electrical Sensors/Voltage Sensor
  + : PMIOPort  Side=Left
  - : PMIOPort  Port=2  Side=Right
  V : Outport
  wires:
  PS-Simulink Converter/1 -> V/1
  connections:
  +/RConn1 -- Voltage Sensor/LConn1
  Voltage Sensor/RConn2 -- -/RConn1
  Voltage Sensor/RConn1 -- PS-Simulink Converter/LConn1

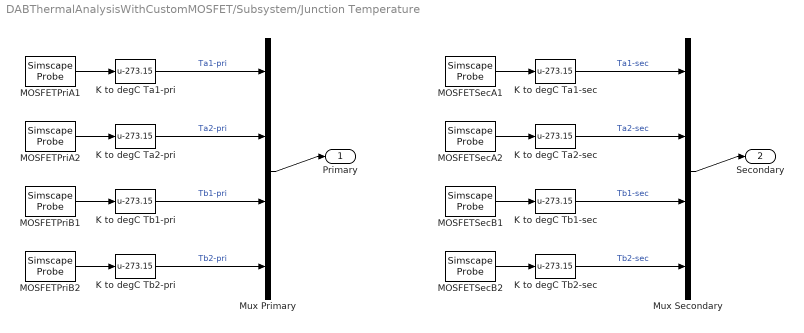
== system DABThermalAnalysisWithCustomMOSFET/Subsystem/Junction Temperature ==
  K to degC Ta1-pri : Bias  Bias=-273.15  SaturateOnIntegerOverflow=off
  K to degC Ta1-sec : Bias  Bias=-273.15  SaturateOnIntegerOverflow=off
  K to degC Ta2-pri : Bias  Bias=-273.15  SaturateOnIntegerOverflow=off
  K to degC Ta2-sec : Bias  Bias=-273.15  SaturateOnIntegerOverflow=off
  K to degC Tb1-pri : Bias  Bias=-273.15  SaturateOnIntegerOverflow=off
  K to degC Tb1-sec : Bias  Bias=-273.15  SaturateOnIntegerOverflow=off
  K to degC Tb2-pri : Bias  Bias=-273.15  SaturateOnIntegerOverflow=off
  K to degC Tb2-sec : Bias  Bias=-273.15  SaturateOnIntegerOverflow=off
  MOSFETPriA1 : SimscapeProbe  BoundBlock=494:1:11190  Variables="{\"T\":{\"Probing\":\"ON\"}}"
  MOSFETPriA2 : SimscapeProbe  BoundBlock=495:1:11190  Variables="{\"T\":{\"Probing\":\"ON\"}}"
  MOSFETPriB1 : SimscapeProbe  BoundBlock=496:1:11190  Variables="{\"T\":{\"Probing\":\"ON\"}}"
  MOSFETPriB2 : SimscapeProbe  BoundBlock=497:1:11190  Variables="{\"T\":{\"Probing\":\"ON\"}}"
  MOSFETSecA1 : SimscapeProbe  BoundBlock=498:585:11190  Variables="{\"T\":{\"Probing\":\"ON\"}}"
  MOSFETSecA2 : SimscapeProbe  BoundBlock=499:585:11190  Variables="{\"T\":{\"Probing\":\"ON\"}}"
  MOSFETSecB1 : SimscapeProbe  BoundBlock=500:585:11190  Variables="{\"T\":{\"Probing\":\"ON\"}}"
  MOSFETSecB2 : SimscapeProbe  BoundBlock=501:585:11190  Variables="{\"T\":{\"Probing\":\"ON\"}}"
  Mux Primary : Mux
  Mux Secondary : Mux
  Primary : Outport
  Secondary : Outport  Port=2
  wires:
  MOSFETPriA1/1 -> K to degC Ta1-pri/1
  K to degC Ta1-pri/1 -> Mux Primary/1  "Ta1-pri"
  MOSFETPriA2/1 -> K to degC Ta2-pri/1
  K to degC Ta2-pri/1 -> Mux Primary/2  "Ta2-pri"
  MOSFETPriB1/1 -> K to degC Tb1-pri/1
  K to degC Tb1-pri/1 -> Mux Primary/3  "Tb1-pri"
  MOSFETPriB2/1 -> K to degC Tb2-pri/1
  K to degC Tb2-pri/1 -> Mux Primary/4  "Tb2-pri"
  Mux Primary/1 -> Primary/1
  MOSFETSecA1/1 -> K to degC Ta1-sec/1
  K to degC Ta1-sec/1 -> Mux Secondary/1  "Ta1-sec"
  MOSFETSecA2/1 -> K to degC Ta2-sec/1
  K to degC Ta2-sec/1 -> Mux Secondary/2  "Ta2-sec"
  MOSFETSecB1/1 -> K to degC Tb1-sec/1
  K to degC Tb1-sec/1 -> Mux Secondary/3  "Tb1-sec"
  MOSFETSecB2/1 -> K to degC Tb2-sec/1
  K to degC Tb2-sec/1 -> Mux Secondary/4  "Tb2-sec"
  Mux Secondary/1 -> Secondary/1

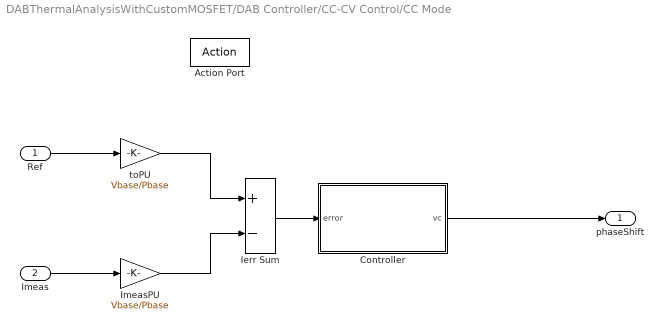
== system DABThermalAnalysisWithCustomMOSFET/DAB Controller/CC-CV Control/CC Mode ==
  Ref : Inport
  Imeas : Inport  Port=2
  Action Port : ActionPort  ActionPortLabel=if(u1 > 0.5)
  Controller : Subsystem  Variant=on  VariantControlMode=label  LabelModeActiveChoice=PIContinuous
  Ierr Sum : Sum  Inputs=+-
  ImeasPU : Gain  Gain=Vbase/Pbase
  toPU : Gain  Gain=Vbase/Pbase
  phaseShift : Outport
  wires:
  Ref/1 -> toPU/1
  toPU/1 -> Ierr Sum/1
  Imeas/1 -> ImeasPU/1
  ImeasPU/1 -> Ierr Sum/2
  Ierr Sum/1 -> Controller/1(error)
  Controller/1(vc) -> phaseShift/1

== system DABThermalAnalysisWithCustomMOSFET/DAB Controller/CC-CV Control/CV Mode ==
  Vref : Inport
  Vmeas : Inport  Port=2
  Action Port : ActionPort  ActionPortLabel=else
  Verr : Sum  Inputs=+-
  Vnorm : Gain  Gain=1/Vbase
  Voltage PI : Subsystem  Variant=on  VariantControlMode=label  LabelModeActiveChoice=PIContinuous
  phaseShift : Outport
  wires:
  Verr/1 -> Vnorm/1
  Vmeas/1 -> Verr/2
  Vref/1 -> Verr/1
  Vnorm/1 -> Voltage PI/1(error)
  Voltage PI/1(vc) -> phaseShift/1

== system DABThermalAnalysisWithCustomMOSFET/DAB Controller/Output Mode/DutyCycle ==
  phaseShift : Inport
  G1 : Outport
  G2 : Outport  Port=2
  wires:
  phaseShift/1 -> G2/1, G1/1

== system DABThermalAnalysisWithCustomMOSFET/DAB Controller/Output Mode/PWMSignal ==
  phaseShift : Inport
  Constant1 : Constant  Value=1/Fsw
  Data Type Conversion : DataTypeConversion  SaturateOnIntegerOverflow=off  RndMeth=Floor
  Data Type Conversion1 : DataTypeConversion  SaturateOnIntegerOverflow=off  RndMeth=Floor
  Gate Signal Generator : Subsystem  AncestorBlock=|
      | eePwmGeneratorTwoLevel/PWM Generator
      | (Three-phase, Two-level)/Gate Signal
      | Generator
  G1 : Outport
  G2 : Outport  Port=2
  wires:
  Constant1/1 -> Gate Signal Generator/1(Ts)
  Gate Signal Generator/2(G2) -> Data Type Conversion1/1
  Gate Signal Generator/1(G1) -> Data Type Conversion/1
  Data Type Conversion/1 -> G1/1
  Data Type Conversion1/1 -> G2/1
  phaseShift/1 -> Gate Signal Generator/2(phaseShift)

== system DABThermalAnalysisWithCustomMOSFET/DAB Converter/Lr/ExternalInductance ==
  Lr : fl_lib/Electrical/Electrical Elements/Inductor  l=DAB.Lr H  r=DAB.RLr Ohm  g=1e-9 1/Ohm  i_specify=off  i_priority=None  i=0 A  i_nominal_specify=off  i_nominal_value=1  i_nominal_unit=A  v_specify=off  v_priority=None  v=0 V  v_nominal_specify=off  v_nominal_value=1  v_nominal_unit=V  i_L_specify=off  i_L_priority=High  i_L=0 A  i_L_nominal_specify=off  i_L_nominal_value=1  i_L_nominal_unit=A
  P : PMIOPort  Side=Left
  N : PMIOPort  Port=2  Side=Right
  connections:
  P/RConn1 -- Lr/LConn1
  Lr/RConn1 -- N/RConn1

== system DABThermalAnalysisWithCustomMOSFET/DAB Controller/CC-CV Control/CC Mode/Controller ==
  error : Inport
  PIContinuous : Subsystem  VariantControl=PIContinuous
  PIDiscrete : Subsystem  VariantControl=PIDiscrete
  vc : Outport

== system DABThermalAnalysisWithCustomMOSFET/DAB Controller/CC-CV Control/CV Mode/Voltage PI ==
  error : Inport
  PIContinuous : Subsystem  VariantControl=PIContinuous
  PIDiscrete : Subsystem  VariantControl=PIDiscrete
  vc : Outport

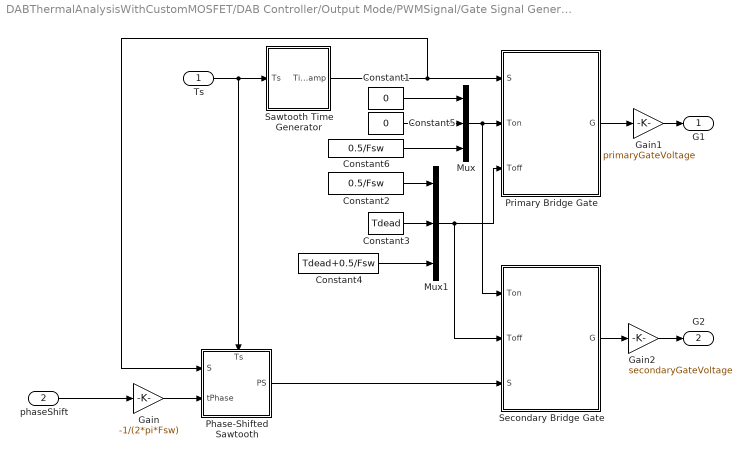
== system DABThermalAnalysisWithCustomMOSFET/DAB Controller/Output Mode/PWMSignal/Gate Signal Generator ==
  Ts : Inport
  phaseShift : Inport  Port=2
  Constant1 : Constant  Value=0
  Constant2 : Constant  Value=0.5/Fsw
  Constant3 : Constant  Value=Tdead
  Constant4 : Constant  Value=Tdead+0.5/Fsw
  Constant5 : Constant  Value=0
  Constant6 : Constant  Value=0.5/Fsw
  Gain : Gain  Gain=-1/(2*pi*Fsw)
  Gain1 : Gain  Gain=primaryGateVoltage
  Gain2 : Gain  Gain=secondaryGateVoltage
  Mux : Mux  Inputs=3
  Mux1 : Mux  Inputs=3
  Phase-Shifted Sawtooth : Subsystem
      settings: PortSchema="{\"entries\":[{\"content\":{\"sides\":[{\"content\":{\"connectorIds\":[\"In1\",\"In2\"]},\"type\":\"ConnectorPlacement.EquallySpacedRectSide\",\"uuid\":\"24147eb6-0623-4755-9b7c-71c26327f18c\"},{\"content\":{\"connectorIds\":[\"Out1\"],\"side\":\"RIGHT\"},\"type\":\"ConnectorPlacement.EquallySpacedRectSide\",\"uuid\":\"2d35ddbe-706c-42fd-ba03-93e64dd64916\"},{\"content\":{\"connectorIds\":[\"In3\"],\"side\":\"TOP\"},\"type\":\"ConnectorPlacement.EquallySpacedRectSide\",\"uuid\":\"9a093734-8ead-449a-8345-ad58ebd72e1a\"}]},\"type\":\"ConnectorPlacement.EquallySpacedConnector\",\"uuid\":\"09c0c51b-93df-4a9e-8785-8511dbaf957c\"}],\"packageUris\":[\"http://schema.mathworks.com/mf0/Connector/R2020b\"],\"version\":\"1.0\"}"
  Primary Bridge Gate : Subsystem
  Sawtooth Time Generator : Subsystem
  Secondary Bridge Gate : Subsystem
  G1 : Outport  VectorParamsAs1DForOutWhenUnconnected=off
  G2 : Outport  Port=2  VectorParamsAs1DForOutWhenUnconnected=off
  wires:
  Phase-Shifted Sawtooth/1(PS) -> Secondary Bridge Gate/3(S)
  Secondary Bridge Gate/1(G) -> Gain2/1
  Primary Bridge Gate/1(G) -> Gain1/1
  Mux1/1 -> Primary Bridge Gate/3(Toff), Secondary Bridge Gate/2(Toff)
  Gain/1 -> Phase-Shifted Sawtooth/2(tPhase)
  Sawtooth Time Generator/1(TimeRamp) -> Primary Bridge Gate/1(S), Phase-Shifted Sawtooth/1(S)
  Constant1/1 -> Mux/1
  Constant5/1 -> Mux/2
  Mux/1 -> Primary Bridge Gate/2(Ton), Secondary Bridge Gate/1(Ton)
  Constant6/1 -> Mux/3
  Constant2/1 -> Mux1/1
  Constant3/1 -> Mux1/2
  Constant4/1 -> Mux1/3
  Ts/1 -> Phase-Shifted Sawtooth/3(Ts), Sawtooth Time Generator/1(Ts)
  phaseShift/1 -> Gain/1
  Gain1/1 -> G1/1
  Gain2/1 -> G2/1

== system DABThermalAnalysisWithCustomMOSFET/DAB Controller/CC-CV Control/CC Mode/Controller/PIContinuous ==
  error : Inport
  PI Controller : slpidlib/PID Controller  Controller=PI  Form=Parallel  TimeDomain=Continuous-time  UseExternalTs=off  SampleTime=-1  IntegratorMethod=Forward Euler  FilterMethod=Forward Euler  ControllerParametersSource=internal  P=Kp  I=Ki  UseKiTs=off  D=0.01  UseExternalDerivativeSource=off  N=100  UseFilter=on  TunerSelectOption=Transfer Function Based (PID Tuner App)  InitialConditionSource=internal  InitialConditionForIntegrator=0  InitialConditionForFilter=0  DifferentiatorICPrevScaledInput=0  ExternalReset=none  TrackingMode=off  Kt=1  LimitOutput=on  SatLimitsSource=internal  UpperSaturationLimit=phaseShiftMax*0.98  LowerSaturationLimit=phaseShiftMin*0.98  LinearizeAsGain=on  AntiWindupMode=clamping  Kb=1  LimitIntegrator=on  UpperIntegratorSaturationLimit=phaseShiftMax*0.98  LowerIntegratorSaturationLimit=phaseShiftMin*0.98  POutMin=[]  POutMax=[]  IOutMin=[]  IOutMax=[]  DOutMin=[]  DOutMax=[]  NOutMin=[]  NOutMax=[]  SumOutMin=[]  SumOutMax=[]  SaturationOutMin=[]  SaturationOutMax=[]  PParamMin=[]  PParamMax=[]  IParamMin=[]  IParamMax=[]  DParamMin=[]  DParamMax=[]  NParamMin=[]  NParamMax=[]  KbParamMin=[]  KbParamMax=[]  KtParamMin=[]  KtParamMax=[]  KbOutMin=[]  KbOutMax=[]  KtOutMin=[]  KtOutMax=[]  IntegratorOutMin=[]  IntegratorOutMax=[]  FilterOutMin=[]  FilterOutMax=[]  SumI1OutMin=[]  SumI1OutMax=[]  SumI2OutMin=[]  SumI2OutMax=[]  SumI3OutMin=[]  SumI3OutMax=[]  SumI4OutMin=[]  SumI4OutMax=[]  SumDOutMin=[]  SumDOutMax=[]  DifferentiatorOutMin=[]  DifferentiatorOutMax=[]  FilterDiffOutCoefMin=[]  FilterDiffOutCoefMax=[]  ReciprocalOutMin=[]  ReciprocalOutMax=[]  SumDenOutMin=[]  SumDenOutMax=[]  SumNumOutMin=[]  SumNumOutMax=[]  DivideOutMin=[]  DivideOutMax=[]  UdiffTsProdOutMin=[]  UdiffTsProdOutMax=[]  NTsProdOutMin=[]  NTsProdOutMax=[]  UintegralTsProdOutMin=[]  UintegralTsProdOutMax=[]  UngainTsProdOutMin=[]  UngainTsProdOutMax=[]  ClampingZeroOutDataTypeStr=Inherit: Inherit via back propagation  ClampingZeroOutMin=[]  ClampingZeroOutMax=[]  FilterDenConstantOutDataTypeStr=Inherit: Inherit via back propagation  FilterDenConstantOutMin=[]  FilterDenConstantOutMax=[]  PCopyOutDataTypeStr=Inherit: Inherit via back propagation  PCopyOutMin=[]  PCopyOutMax=[]  NCopyOutDataTypeStr=Inherit: Inherit via back propagation  NCopyOutMin=[]  NCopyOutMax=[]  IntegratorContinuousStateAttributes=''  IntegratorStateMustResolveToSignalObject=off  IntegratorRTWStateStorageClass=Auto  FilterContinuousStateAttributes=''  FilterStateMustResolveToSignalObject=off  FilterRTWStateStorageClass=Auto  ParallelPVariant=InternalParameters  IdealPVariant=Disabled  IVariant=InternalParameters  DVariant=Disabled  IntegratorVariant=Continuous  SatVariant=Enabled  AWVariant=ContClampingParallel  PCopyVariant=Disabled  TRVariant=Disabled  FdbkBlocksVariant=Forward  IdealPFdbkVariant=Disabled  SatFdbkVariant=Disabled  DerivativeFilterVariant=Disabled  NVariant=Disabled  NCopyVariant=Disabled_SignalSpec  FilterICVariant=Disabled  IntegratorICVariant=InternalICs  ExternalResetVariant=Disabled  TRSumVariant=Passthrough  SumFdbkVariant=Disabled  SumVariant=Sum_PI  TsampFilterVariant=InternalTs  TsampNgainVariant=Passthrough  TsampIntegralVariant=Disabled_SignalSpec  ExternalSaturationOutDataTypeStr=Inherit: Same as second input  DerivativeSourceVariant=Disabled  PreIntVariant=InternalPreInt
  vc : Outport
  wires:
  error/1 -> PI Controller/1
  PI Controller/1 -> vc/1

== system DABThermalAnalysisWithCustomMOSFET/DAB Controller/CC-CV Control/CC Mode/Controller/PIDiscrete ==
  error : Inport
  PI Controller : slpidlib/PID Controller  Controller=PI  Form=Parallel  TimeDomain=Discrete-time  UseExternalTs=off  SampleTime=Ts  IntegratorMethod=Forward Euler  FilterMethod=Forward Euler  ControllerParametersSource=internal  P=Kp  I=Ki  UseKiTs=off  D=0  UseExternalDerivativeSource=off  N=100  UseFilter=on  TunerSelectOption=Transfer Function Based (PID Tuner App)  InitialConditionSource=internal  InitialConditionForIntegrator=0  InitialConditionForFilter=0  DifferentiatorICPrevScaledInput=0  ExternalReset=none  TrackingMode=off  Kt=1  LimitOutput=on  SatLimitsSource=internal  UpperSaturationLimit=phaseShiftMax  LowerSaturationLimit=phaseShiftMin  LinearizeAsGain=on  AntiWindupMode=clamping  Kb=1  LimitIntegrator=on  UpperIntegratorSaturationLimit=phaseShiftMax  LowerIntegratorSaturationLimit=phaseShiftMin  POutMin=[]  POutMax=[]  IOutMin=[]  IOutMax=[]  DOutMin=[]  DOutMax=[]  NOutMin=[]  NOutMax=[]  SumOutMin=[]  SumOutMax=[]  SaturationOutMin=[]  SaturationOutMax=[]  PParamMin=[]  PParamMax=[]  IParamMin=[]  IParamMax=[]  DParamMin=[]  DParamMax=[]  NParamMin=[]  NParamMax=[]  KbParamMin=[]  KbParamMax=[]  KtParamMin=[]  KtParamMax=[]  KbOutMin=[]  KbOutMax=[]  KtOutMin=[]  KtOutMax=[]  IntegratorOutMin=[]  IntegratorOutMax=[]  FilterOutMin=[]  FilterOutMax=[]  SumI1OutMin=[]  SumI1OutMax=[]  SumI2OutMin=[]  SumI2OutMax=[]  SumI3OutMin=[]  SumI3OutMax=[]  SumI4OutMin=[]  SumI4OutMax=[]  SumDOutMin=[]  SumDOutMax=[]  DifferentiatorOutMin=[]  DifferentiatorOutMax=[]  FilterDiffOutCoefMin=[]  FilterDiffOutCoefMax=[]  ReciprocalOutMin=[]  ReciprocalOutMax=[]  SumDenOutMin=[]  SumDenOutMax=[]  SumNumOutMin=[]  SumNumOutMax=[]  DivideOutMin=[]  DivideOutMax=[]  UdiffTsProdOutMin=[]  UdiffTsProdOutMax=[]  NTsProdOutMin=[]  NTsProdOutMax=[]  UintegralTsProdOutMin=[]  UintegralTsProdOutMax=[]  UngainTsProdOutMin=[]  UngainTsProdOutMax=[]  ClampingZeroOutDataTypeStr=Inherit: Inherit via back propagation  ClampingZeroOutMin=[]  ClampingZeroOutMax=[]  FilterDenConstantOutDataTypeStr=Inherit: Inherit via back propagation  FilterDenConstantOutMin=[]  FilterDenConstantOutMax=[]  PCopyOutDataTypeStr=Inherit: Inherit via back propagation  PCopyOutMin=[]  PCopyOutMax=[]  NCopyOutDataTypeStr=Inherit: Inherit via back propagation  NCopyOutMin=[]  NCopyOutMax=[]  IntegratorContinuousStateAttributes=''  IntegratorStateMustResolveToSignalObject=off  IntegratorRTWStateStorageClass=Auto  FilterContinuousStateAttributes=''  FilterStateMustResolveToSignalObject=off  FilterRTWStateStorageClass=Auto  ParallelPVariant=InternalParameters  IdealPVariant=Disabled  IVariant=InternalParameters  DVariant=Disabled  IntegratorVariant=Discrete  SatVariant=Enabled  AWVariant=DiscClampingParallel  PCopyVariant=Disabled  TRVariant=Disabled  FdbkBlocksVariant=Forward  IdealPFdbkVariant=Disabled  SatFdbkVariant=Disabled  DerivativeFilterVariant=Disabled  NVariant=Disabled  NCopyVariant=Disabled_SignalSpec  FilterICVariant=Disabled  IntegratorICVariant=InternalICs  ExternalResetVariant=Disabled  TRSumVariant=Passthrough  SumFdbkVariant=Disabled  SumVariant=Sum_PI  TsampFilterVariant=InternalTs  TsampNgainVariant=Passthrough  TsampIntegralVariant=Disabled_SignalSpec  ExternalSaturationOutDataTypeStr=Inherit: Same as second input  DerivativeSourceVariant=Disabled  PreIntVariant=InternalPreInt
  vc : Outport
  wires:
  error/1 -> PI Controller/1
  PI Controller/1 -> vc/1
